simulink model "aircraft_6dof_cl"  (R2025b)
settings: Solver=VariableStepAuto  StartTime=0.0  StopTime=10  FixedStep=0.01  RelTol=1e-3
InitFcn:
  | trim_cl
values from neighbouring files (symbols this model uses):
  alpha0 = fzero(@(a) trimResidual(a, mach0, q, W, CDair), [0 10])    [trim_cl.m]
  CDair = 0.02    [trim_cl.m]
  CM0 = y(3)    [trim_cl.m]
  T0 = D / cosd(alpha0)    [trim_cl.m]
  theta0 = alpha0 * pi / 180    [trim_cl.m]
  u0 = V0 * cosd(alpha0)    [trim_cl.m]
  w0 = V0 * sind(alpha0)    [trim_cl.m]
settings Model: Creator=HP  LastModifiedBy=HP

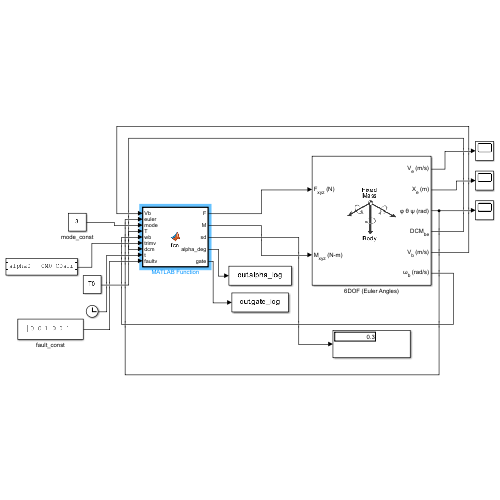
[thumbnail: Simulink's stored preview of the top-level diagram]
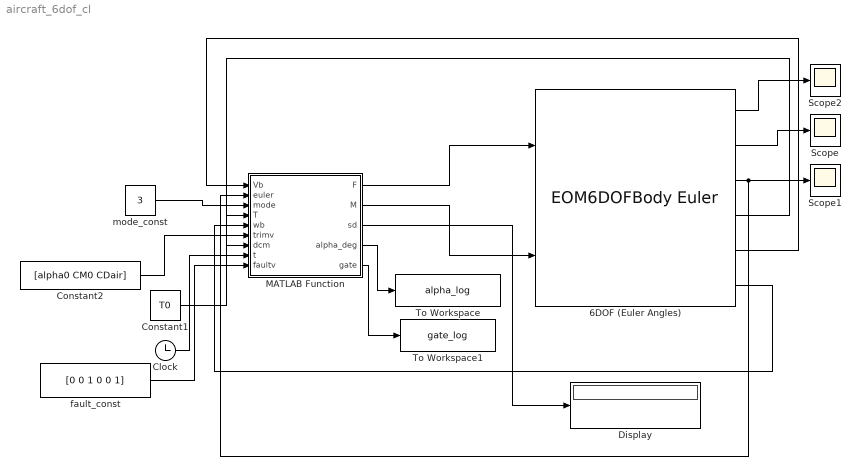
== system aircraft_6dof_cl ==
  6DOF (Euler Angles) : EOM6DOFBodyEuler  Vm_0=[u0 0 w0]  eul_0=[0 theta0 0]  mass_0=5
  Clock : Clock
  Constant1 : Constant  Value=T0
  Constant2 : Constant  Value=[alpha0 CM0 CDair]
  Display : Display
  MATLAB Function : MATLAB Function  TreatAsAtomicUnit=on
  Scope : Scope
      settings: ActiveDisplayYMinimum=-1  ActiveDisplayYMaximum=1  DataLoggingVariableName=log_Scope
  Scope1 : Scope
      settings: ActiveDisplayYMinimum=-1  ActiveDisplayYMaximum=1  DataLoggingVariableName=log_Scope1
  Scope2 : Scope
      settings: ActiveDisplayYMinimum=-1  ActiveDisplayYMaximum=1  DataLoggingVariableName=log_Scope2
  To Workspace : ToWorkspace  VariableName=alpha_log  SaveFormat=Structure With Time  SampleTime=-1
  To Workspace1 : ToWorkspace  VariableName=gate_log  SaveFormat=Structure With Time  SampleTime=-1
  fault_const : Constant  Value=[0 0 1 0 0 1]
  mode_const : Constant  Value=3
  wires:
  6DOF (Euler Angles)/2 -> Scope/1
  6DOF (Euler Angles)/1 -> Scope2/1
  6DOF (Euler Angles)/3 -> MATLAB Function/2(euler), Scope1/1
  MATLAB Function/1(F) -> 6DOF (Euler Angles)/1
  MATLAB Function/2(M) -> 6DOF (Euler Angles)/2
  MATLAB Function/3(sd) -> Display/1
  mode_const/1 -> MATLAB Function/3(mode)
  6DOF (Euler Angles)/5 -> MATLAB Function/1(Vb)
  Constant1/1 -> MATLAB Function/4(T)
  6DOF (Euler Angles)/6 -> MATLAB Function/5(wb)
  Constant2/1 -> MATLAB Function/6(trimv)
  6DOF (Euler Angles)/4 -> MATLAB Function/7(dcm)
  Clock/1 -> MATLAB Function/8(t)
  fault_const/1 -> MATLAB Function/9(faultv)
  MATLAB Function/4(alpha_deg) -> To Workspace/1
  MATLAB Function/5(gate) -> To Workspace1/1

== matlab function aircraft_6dof_cl/MATLAB Function ==
  data: Vb input; euler input; F output; M output; sd output; mode input; T input; alpha_deg output; wb input; trimv input; dcm input; t input; faultv input; gate output
function [F, M, sd, alpha_deg, gate] = fcn(Vb, euler, mode, T, wb, trimv, dcm, t, faultv)
coder.extrinsic('gp_predict_flight');
coder.extrinsic('lookup_predict');
coder.extrinsic('truth_predict');

% Aircraft numbers (docs/aircraft_assumptions.md)
rho  = 1.225;   % air density, kg/m3
S    = 0.15;    % wing area, m2
c    = 0.3;     % chord, m
mass = 5;       % kg
g    = 9.81;    % m/s2

% Illustrative tail (not real tail aerodynamics)
Cma = -0.5;     % restoring moment per radian of angle away from trim
Cmq = -10;      % pitch damping

alpha0 = trimv(1) * pi / 180;   % trim angle of attack, rad
CM0    = trimv(2);              % airfoil CM at trim (balanced by the tail)
CDair  = trimv(3);              % extra airframe drag (same in all modes)

% Training data box of the flight GP (docs/range_rule_rules.md)
aMin = -5;  aMax = 15;          % alpha, deg
mMin = 0;   mMax = 0.4;         % Mach

% ---- Faults (docs/fault_test_rules.md) ----
% faultv = [gust peak (m/s), gust start (s), gust duration (s), fault max dCm, fault start (s), fault ramp time (s)]
wg = 0;
if t >= faultv(2) && t <= faultv(2) + faultv(3)
    wg = faultv(1) / 2 * (1 - cos(2 * pi * (t - faultv(2)) / faultv(3)));   % 1-cos upward gust
end
dCm = 0;
if t >= faultv(5)
    dCm = faultv(4) * min(1, (t - faultv(5)) / faultv(6));                    % slow nose-up trim runaway
end

% ---- Airflow relative to the air (body axes: x forward, z down) ----
wind_e = [0; 0; -wg];                % upward gust in Earth axes (NED: up is -z)
wind_b = dcm * wind_e;               % gust in body axes
Va = Vb(:) - wind_b;                 % air-relative velocity
u = Va(1);  v = Va(2);  w = Va(3);
V = sqrt(u^2 + v^2 + w^2);           % airspeed, m/s
V = max(V, 1);                       % avoid dividing by zero
alpha = atan2(w, u);                 % angle of attack, rad
alpha_deg = alpha * 180 / pi;
mach = V / 340;

% ---- Coefficients from the chosen source ----
yg  = zeros(1,3);
yl  = zeros(1,3);
yt  = zeros(1,3);
sd  = 0;
thr = 0;
[yg, sd, thr] = gp_predict_flight(alpha_deg, mach);
yl = lookup_predict(alpha_deg, mach);

inBox = alpha_deg >= aMin && alpha_deg <= aMax && mach >= mMin && mach <= mMax;

y = yl;                              % mode 1: lookup only
gate = 0;                            % 1 when the GP is used
if mode == 0
    yt = truth_predict(alpha_deg, mach);
    y = yt;                          % mode 0: truth (reference)
elseif mode == 2
    y = yg;                          % mode 2: GP only
    gate = 1;
elseif mode == 3 && sd <= thr
    y = yg;                          % mode 3: GP when sure, else lookup
    gate = 1;
elseif mode == 4 && inBox
    y = yg;                          % mode 4: GP inside the training data box, else lookup
    gate = 1;
end

% ---- Aerodynamic forces, turned into body axes ----
qbar = 0.5 * rho * V^2 * S;
L = qbar * y(1);
D = qbar * (y(2) + CDair);
Xa = -D * cos(alpha) + L * sin(alpha);
Za = -D * sin(alpha) - L * cos(alpha);

% ---- Gravity in body axes (uses roll and pitch) ----
phi = euler(1);  theta = euler(2);
Fg = mass * g * [-sin(theta); sin(phi) * cos(theta); cos(phi) * cos(theta)];

F = [Xa + T; 0; Za] + Fg;

% ---- Pitching moment: airfoil CM + illustrative tail + trim fault ----
qrate = wb(2);                       % pitch rate, rad/s
Cm = (y(3) - CM0) + Cma * (alpha - alpha0) + Cmq * qrate * c / (2 * V) + dCm;
M = [0; qbar * c * Cm; 0];
end
